simulink model "tanque_hil_mil_2021a"  (R2023b)
settings: Solver=VariableStepAuto  StartTime=0.0  StopTime=300  FixedStep=0.001  RelTol=1e-4
values from neighbouring files (symbols this model uses):
  Cz = tf(Cz)    [controlar_tanque.m]    (also in pidtune.m)
undefined symbols (not defined in the file or in its folder): LF
libraries: instrumentseriallib x3, svdutilitieslib x1
settings Model: Creator=tom  LastModifiedBy=fjmoy
settings DebuggingCC: SignalInfNanChecking=warning  UnconnectedInputMsg=warning  UnconnectedOutputMsg=warning  UnconnectedLineMsg=warning
settings ModelReferenceCC: EnableRefExpFcnMdlSchedulingChecks=on
settings RTWCC: DLArmComputeVersion=19.05

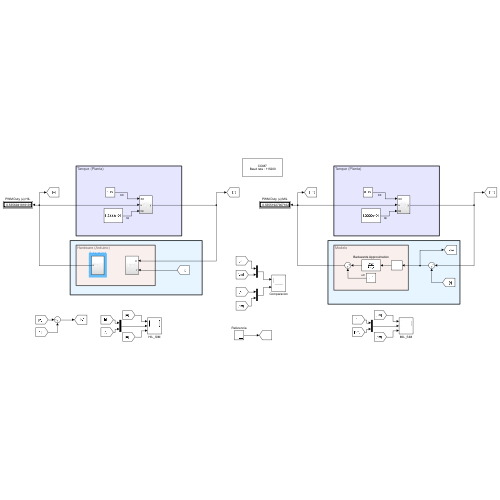
[thumbnail: Simulink's stored preview of the top-level diagram]
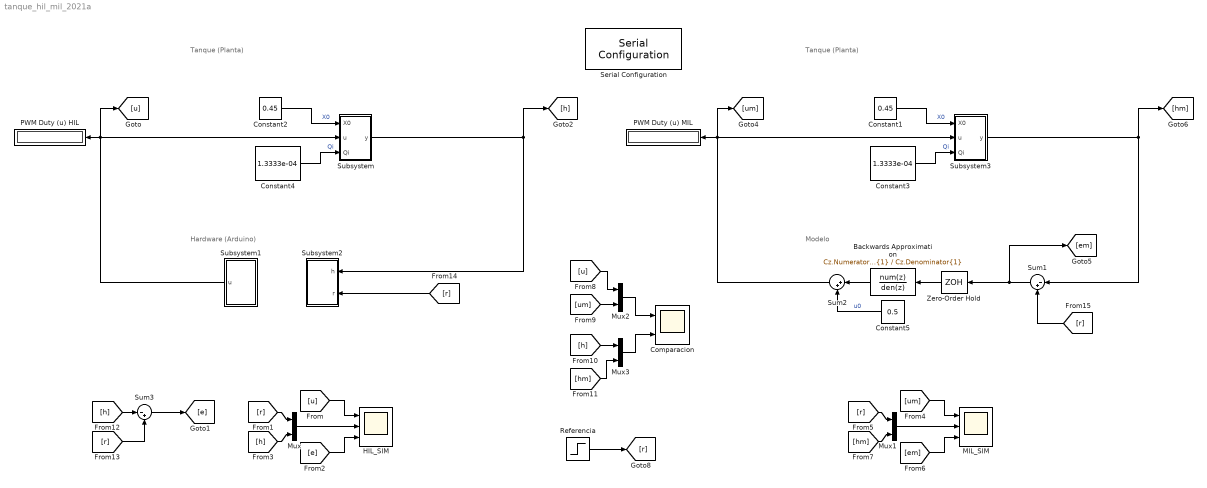
== system tanque_hil_mil_2021a ==
  note: Hardware (Arduino)
  note: Tanque (Planta)
  note: Tanque (Planta)
  note: Modelo
  Backwards Approximation : DiscreteTransferFcn  Numerator=Cz.Numerator{1}  Denominator=Cz.Denominator{1}  SampleTime=1  a0EqualsOne=on  StateName=C_for
  Comparacion : Scope  NumInputPorts=2
  Constant1 : Constant  Value=0.45
  Constant2 : Constant  Value=0.45
  Constant3 : Constant  Value=1.3333e-04
  Constant4 : Constant  Value=1.3333e-04
  Constant5 : Constant  Value=0.5
  HIL_SIM : Scope  NumInputPorts=3
  MIL_SIM : Scope  NumInputPorts=3
  Mux{,1..3} (4 alike) : Mux  Inputs=2
  PWM Duty (u) HIL : Display
      settings: Format=decimal (Stored Integer)
  PWM Duty (u) MIL : Display
      settings: Format=decimal (Stored Integer)
  Referencia : Step  Time=0  Before=0.45  After=0.4  SampleTime=0
  Serial Configuration : instrumentseriallib/Serial Configuration  Priority=-200000  PortSel=COM7  Port=COM7  ComPort=COM7  BaudRate=115200  DataBits=8  Parity=none  StopBits=1  ByteOrder=little-endian  FlowControl=none  Timeout=10  SimulateUsing=Interpreted execution  BlockInModel=on  aMode=1
  Subsystem : Subsystem
  Subsystem1 : Subsystem
  Subsystem2 : Subsystem
  Subsystem3 : Subsystem
  Sum1 : Sum  Inputs=|-+
  Sum2 : Sum  Inputs=|++
  Sum3 : Sum  Inputs=|-+
  Zero-Order Hold : ZeroOrderHold
  wires:
  Constant2/1 -> Subsystem/1(X0)  "X0"
  Constant4/1 -> Subsystem/3(Qi)  "Qi"
  Subsystem1/1(u) -> [u], PWM Duty (u) HIL/1, Subsystem/2(u)
  Subsystem/1(y) -> Subsystem2/1(h), [h]
  [u] -> HIL_SIM/1
  Mux/1 -> HIL_SIM/2
  [e] -> HIL_SIM/3
  [r] -> Mux/1
  [h] -> Mux/2
  Subsystem3/1(y) -> [hm], Sum1/1
  [em] -> MIL_SIM/3
  [um] -> MIL_SIM/1
  Mux1/1 -> MIL_SIM/2
  [r] -> Mux1/1
  Constant1/1 -> Subsystem3/1(X0)  "X0"
  [hm] -> Mux1/2
  Constant3/1 -> Subsystem3/3(Qi)  "Qi"
  Constant5/1 -> Sum2/2  "u0"
  Sum2/1 -> [um], PWM Duty (u) MIL/1, Subsystem3/2(u)
  Sum1/1 -> Zero-Order Hold/1, [em]
  Zero-Order Hold/1 -> Backwards Approximation/1
  Mux2/1 -> Comparacion/1
  [u] -> Mux2/1
  [um] -> Mux2/2
  [h] -> Mux3/1
  [hm] -> Mux3/2
  Mux3/1 -> Comparacion/2
  [h] -> Sum3/1
  Sum3/1 -> [e]
  [r] -> Sum3/2
  Referencia/1 -> [r]
  [r] -> Subsystem2/2(r)
  [r] -> Sum1/2
  Backwards Approximation/1 -> Sum2/1

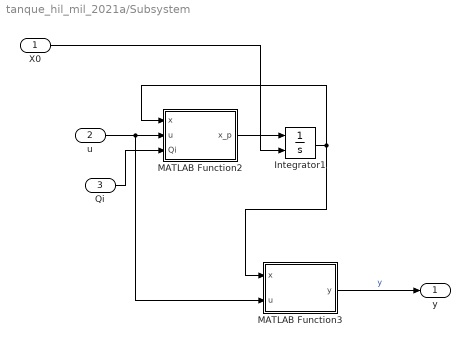
== system tanque_hil_mil_2021a/Subsystem ==
  X0 : Inport
  u : Inport  Port=2
  Qi : Inport  Port=3
  Integrator1 : Integrator  InitialConditionSource=external
  MATLAB Function2 : MATLAB Function  TreatAsAtomicUnit=on
  MATLAB Function3 : MATLAB Function  TreatAsAtomicUnit=on
  y : Outport
  wires:
  X0/1 -> Integrator1/2
  Integrator1/1 -> MATLAB Function3/1(x), MATLAB Function2/1(x)
  u/1 -> MATLAB Function3/2(u), MATLAB Function2/2(u)
  MATLAB Function2/1(x_p) -> Integrator1/1
  MATLAB Function3/1(y) -> y/1  "y"
  Qi/1 -> MATLAB Function2/3(Qi)

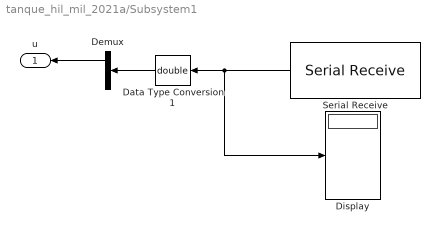
== system tanque_hil_mil_2021a/Subsystem1 ==
  Data Type Conversion1 : DataTypeConversion  OutDataTypeStr=double  SaturateOnIntegerOverflow=off  RndMeth=Floor
  Demux : Demux  Outputs=3
  Display : Display
      settings: Format=decimal (Stored Integer)
  Serial Receive : instrumentseriallib/Serial Receive  PortSel=COM7  Port=COM7  ComPort=COM7  DataType=single  SaveDataType=uint8  ToggleHeader=on  Header="[ 97   98   99  100 ]"  ToggleTerminator=off  Terminator=LF ('\n')  CustomTerminator=[]  InputFormat=Column major  ToggleDataSize=on  DataSize=[3 1]  EnableBlockingMode=on  ActionDataUnavailable=Output custom value  ActionWhenDataUnavailable=Output custom value  CustomValue=0.5  SampleTime=1  SimulateUsing=Interpreted execution  BlockInModel=on  aMode=1
  u : Outport
  wires:
  Serial Receive/1 -> Display/1, Data Type Conversion1/1
  Data Type Conversion1/1 -> Demux/1
  Demux/1 -> u/1

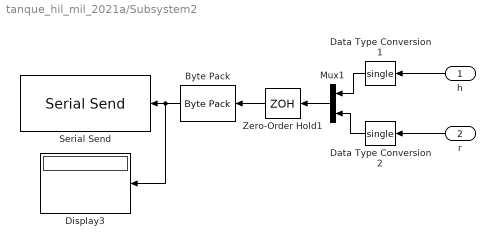
== system tanque_hil_mil_2021a/Subsystem2 ==
  h : Inport
  r : Inport  Port=2
  Byte Pack : svdutilitieslib/Byte Pack  maskPackedDataType=uint32  datatypes={'single'}  byteAlign=4  blockPlatform=arduinoert
  Data Type Conversion1 : DataTypeConversion  OutDataTypeStr=single  SaturateOnIntegerOverflow=off  RndMeth=Floor
  Data Type Conversion2 : DataTypeConversion  OutDataTypeStr=single  SaturateOnIntegerOverflow=off  RndMeth=Floor
  Display3 : Display
      settings: Format=hex (Stored Integer)
  Mux1 : Mux  Inputs=2
  Serial Send : instrumentseriallib/Serial Send  PortSel=COM7  Port=COM7  ComPort=COM7  Header=[65, 66, 67, 68]  Terminator=<none>  CustomTerminator=[]  EnableBlockingMode=on  SimulateUsing=Interpreted execution  BlockInModel=on  aMode=1
  Zero-Order Hold1 : ZeroOrderHold
  wires:
  h/1 -> Data Type Conversion1/1
  Byte Pack/1 -> Display3/1, Serial Send/1
  Zero-Order Hold1/1 -> Byte Pack/1
  Mux1/1 -> Zero-Order Hold1/1
  Data Type Conversion2/1 -> Mux1/2
  Data Type Conversion1/1 -> Mux1/1
  r/1 -> Data Type Conversion2/1

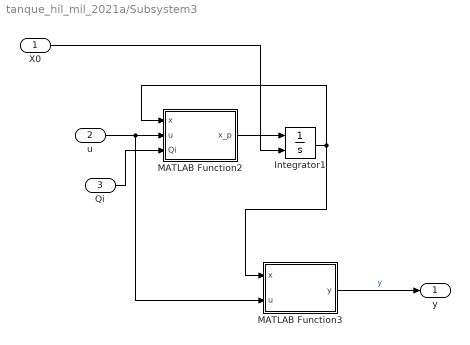
== system tanque_hil_mil_2021a/Subsystem3 ==
  X0 : Inport
  u : Inport  Port=2
  Qi : Inport  Port=3
  Integrator1 : Integrator  InitialConditionSource=external
  MATLAB Function2 : MATLAB Function  TreatAsAtomicUnit=on
  MATLAB Function3 : MATLAB Function  TreatAsAtomicUnit=on
  y : Outport
  wires:
  X0/1 -> Integrator1/2
  Integrator1/1 -> MATLAB Function3/1(x), MATLAB Function2/1(x)
  u/1 -> MATLAB Function3/2(u), MATLAB Function2/2(u)
  MATLAB Function2/1(x_p) -> Integrator1/1
  MATLAB Function3/1(y) -> y/1  "y"
  Qi/1 -> MATLAB Function2/3(Qi)

== matlab function tanque_hil_mil_2021a/Subsystem3/MATLAB Function2 ==
  data: x input size=1; u input size=1; x_p output size=1; Qi input
function x_p = f(x, u, Qi)
    d = 0.01065;
    L1 = 0.1;
    L2 = 0.4;
    L = 0.9;
    g = 9.8;
    x_p = (-sqrt(abs(2*g*x))*d^2/4*u*pi + Qi)/(L1+(L2-L1)*x/L)^2;

== matlab function tanque_hil_mil_2021a/Subsystem3/MATLAB Function3 ==
  data: x input; u input; y output
function y = g(x, u)
    y = x;

== matlab function tanque_hil_mil_2021a/Subsystem/MATLAB Function3 ==
  data: x input; u input; y output
function y = g(x, u)
    y = x;

== matlab function tanque_hil_mil_2021a/Subsystem/MATLAB Function2 ==
  data: x input size=1; u input size=1; x_p output size=1; Qi input
function x_p = f(x, u, Qi)
    d = 0.01065;
    L1 = 0.1;
    L2 = 0.4;
    L = 0.9;
    g = 9.8;
    x_p = (-sqrt(abs(2*g*x))*d^2/4*u*pi + Qi)/(L1+(L2-L1)*x/L)^2;
